simulink model "Copy_of_model"  (R2015a)
settings: Solver=ode3  StartTime=0.0  StopTime=200  RelTol=1e-3
undefined symbols (not defined in the file): MIO, National_Instruments, PCI
libraries: sldrtlib x3
settings Model: SimulationMode=external  ExtModeTrigDuration=200001  Creator=Alunos  LastModifiedBy=Alunos
settings HardwareCC: ProdIntDivRoundTo=Zero  ProdEndianess=LittleEndian  ProdHWDeviceType=Intel->x86/Pentium  TargetIntDivRoundTo=Zero  TargetEndianess=LittleEndian  TargetHWDeviceType=Intel->x86/Pentium
settings RTWCC: SystemTargetFile=rtwin.tlc  TemplateMakefile=rtwin.tmf  Description=Simulink Desktop Real-Time  RTWCompilerOptimization=on
settings CodeAppCC: MaxIdLength=95
settings RTWinTargetCC: TargetPreCompLibLocation=C:\Program Files\MATLAB\R2015a\toolbox\sldrt\lib\win32

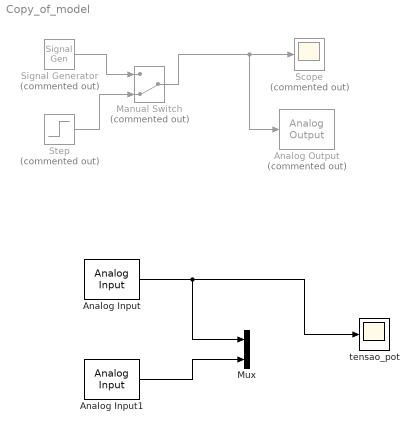
== system Copy_of_model ==
  Analog Input : sldrtlib/Analog Input  SampleTime=0.001  MaxMissedTicks=10  ShowMissedTicks=off  YieldWhenWaiting=off  DrvName=National_Instruments/PCI-MIO-16E-4  DrvAddress=4294967295  DrvOptions=[0 0 0 0 0 0]  Channels=1:2  RangeMode=1  VoltRange=1  DataType=1
      settings: AttributesFormatString=National Instruments\nPCI-MIO-16E-4 [auto]
  Analog Input1 : sldrtlib/Analog Input  SampleTime=0.001  MaxMissedTicks=10  ShowMissedTicks=off  YieldWhenWaiting=off  DrvName=National_Instruments/PCI-MIO-16E-4  DrvAddress=4294967295  DrvOptions=[0 0 0 0 0 0]  Channels=1  RangeMode=1  VoltRange=1  DataType=1
      settings: AttributesFormatString=National Instruments\nPCI-MIO-16E-4 [auto]
  Analog Output : sldrtlib/Analog Output  Commented=on  SampleTime=0.001  MaxMissedTicks=10  ShowMissedTicks=off  YieldWhenWaiting=off  DrvName=National_Instruments/PCI-MIO-16E-4  DrvAddress=4294967295  DrvOptions=[0 0 0 0 0 0]  Channels=1  RangeMode=1  VoltRange=1  InitialValue=0  FinalValue=0
      settings: AttributesFormatString=National Instruments\nPCI-MIO-16E-4 [auto]
  Manual Switch : ManualSwitch  Commented=on  CurrentSetting=0
  Mux : Mux  Inputs=2
  Scope : Scope  Commented=on
      settings: TickLabels=on  SaveName=input  SampleInput=on  SampleTime=0.001
  Signal Generator : SignalGenerator  Commented=on  WaveForm=square  Amplitude=2
  Step : Step  Commented=on  SampleTime=0.001
  "tensao_pot " : Scope
      settings: TickLabels=on  YMin=-4.5  YMax=2  SaveName=tensao_pot  SampleInput=on  SampleTime=0.001
  wires:
  Manual Switch/1 -> Analog Output/1, Scope/1
  Signal Generator/1 -> Manual Switch/1
  Step/1 -> Manual Switch/2
  Analog Input1/1 -> Mux/2
  Analog Input/1 -> "tensao_pot "/1, Mux/1
